simulink model "simulink_flightgear_control_trim_wind_5"  (R2023a)
settings: Solver=VariableStepAuto  StartTime=0  StopTime=inf  FixedStep=0.1  RelTol=1e-3
values from neighbouring files (symbols this model uses):
  alpha = -5:0.1:25    [Boeing747model.m]
  alpha1 = 0:0.1:14    [Boeing747model.m]
  alpha2 = -5:0.1:25    [Boeing747model.m]
  alpha3 = -5:0.1:17    [Boeing747model.m]
  beta = -15:0.1:15    [Boeing747model.m]
  CL = 0:0.01:1.4    [Boeing747model.m]
  da = 0:1:20    [Boeing747model.m]
  dr = [0 5 10 15 20 25]    [Boeing747model.m]
  EPR_ = 0:0.1:1.8    [Boeing747model.m]    (also in engine.m)
  flap = [0 10 20 25 30]    [Boeing747model.m]
  high1 = 0:10000:40000    [Boeing747model.m]
  high2 = 0:20000:40000    [Boeing747model.m]
  high3 = [0 15000 25000 35000 40000]    [Boeing747model.m]    (also in engine.m)
  high4 = [0 10000 20000 40000]    [Boeing747model.m]
  interp_result = table2array(resultTable(:,2:end))    [Boeing747model.m]
  interp_result_mach = 0:0.1:0.9    [Boeing747model.m]
  interp_result_N1 = 80:5:110    [Boeing747model.m]
  m2ft = 3.280839895013    (= 3.28083989501)    [Boeing747model.m]    (also in engine.m)
  mach = 0:0.02:0.9    [Boeing747model.m]    (also in engine.m)
  mach1 = [0 0.3 0.5 0.7 0.8 0.84 0.86 0.88 0.9]    [Boeing747model.m]
  mach2 = [0 0.3 0.5 0.7 0.8 0.9]    [Boeing747model.m]
  mach3 = [0 0.1 0.3 0.5 0.6 0.7 0.8 0.9]    [Boeing747model.m]    (also in engine.m = [0 0.1 0.3 0.5  0.7 0.8 0.9])
  mach5 = [0 0.6 0.8 0.85 0.9]    [Boeing747model.m]
  mach6 = [0 0.6 0.8 0.9]    [Boeing747model.m]
  mach7 = [0 0.3 0.5 0.74 0.8 0.84 0.86 0.88 0.9]    [Boeing747model.m]
  mach8 = [0 0.3 0.5 0.74 0.8 0.84 0.86 0.88 0.9]    [Boeing747model.m]
  model = 'simulink_flightgear_control_trim_wind_5'    [traimcode.m]
  ms2kts = 1.943844492609    (= 1.94384449261)    [Boeing747model.m]    (also in engine.m)
  powerangle_ = 0:1:130    [Boeing747model.m]    (also in engine.m)
  T = [-45 0 60 120]    [Boeing747model.m]    (also in engine.m)
  V_E = 0:20:250    [Boeing747model.m]
undefined symbols (not defined in the file or in its folder): Earth, F, ft, Light, m, MIL, Model, Newton, P3DAERO, Raphson, Receive, s, Send, Unit, WGS84, Wind
libraries: simulink_extras x115, aerolibconvert2 x16, simulink x4, aerolibfltsims x3, shared6dof x1, aerolibasang x1, aerolibtransform2 x1, aerolibatmos2 x1, aerolibobsolete x1, aerolibwind2 x1
(part 2 of 5)

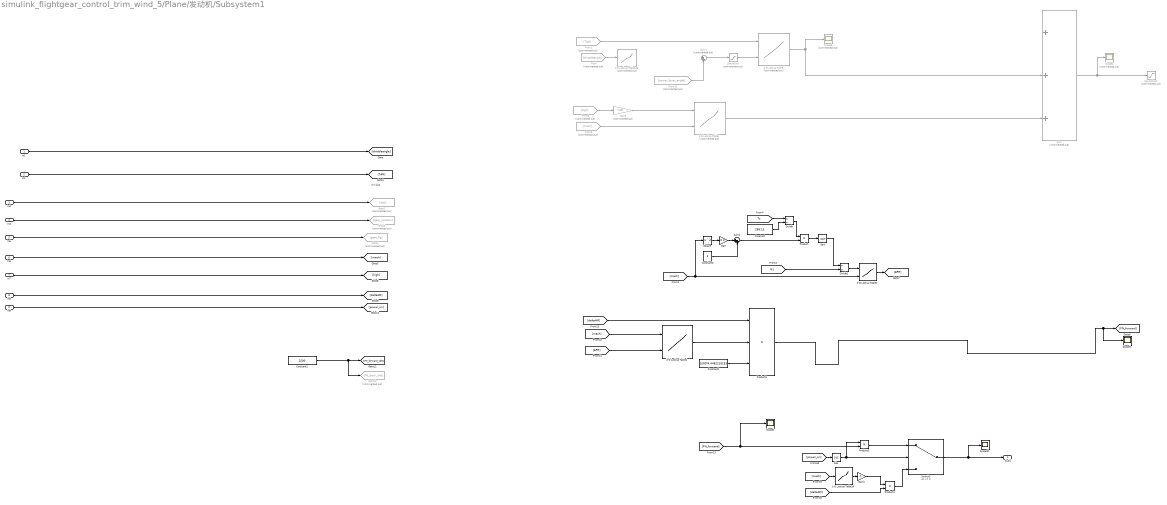
== system simulink_flightgear_control_trim_wind_5/Plane/发动机/Subsystem1 ==
  note: 华氏温度
  In1 : Inport
  In2 : Inport  Port=2
  In3 : Inport  Port=3
  In4 : Inport  Port=4
  In5 : Inport  Port=5
  In6 : Inport  Port=6
  In7 : Inport  Port=7
  In8 : Inport  Port=8
  In9 : Inport  Port=9
  1-D Lookup Table106 : Lookup_n-D  Commented=on  NumberOfTableDimensions=1  BreakpointsForDimension1=P3DAERO.powerangle(1,:)  Table=P3DAERO.powerangle(2,:)  InternalRulePriority=Speed  RndMeth=Simplest
  1-D Lookup Table14 : Lookup_n-D  NumberOfTableDimensions=1  BreakpointsForDimension1=P3DAERO.FD_engine(1,:)  Table=P3DAERO.FD_engine(2,:)  InternalRulePriority=Speed  RndMeth=Simplest
  2-D Lookup Table : Lookup_n-D  Commented=on  BreakpointsForDimension1=T  BreakpointsForDimension2=powerangle_  Table=P3DAERO.tam  InternalRulePriority=Speed  RndMeth=Simplest
      settings: InputPortMap=u0,u1
  2-D Lookup Table1 : Lookup_n-D  Commented=on  BreakpointsForDimension1=high3  BreakpointsForDimension2=mach  Table=P3DAERO.EPR_decay  InternalRulePriority=Speed  RndMeth=Simplest
      settings: InputPortMap=u0,u1
  2-D Lookup Table2 : Lookup_n-D  BreakpointsForDimension1=interp_result_N1  BreakpointsForDimension2=interp_result_mach  Table=interp_result  InternalRulePriority=Speed  RndMeth=Simplest
      settings: InputPortMap=u0,u1
  2-D Lookup Table4 : Lookup_n-D  BreakpointsForDimension1=mach3  BreakpointsForDimension2=EPR_  Table=P3DAERO.FN_deltaAM  InternalRulePriority=Speed  RndMeth=Simplest
      settings: InputPortMap=u0,u1
  Abs : Abs  SaturateOnIntegerOverflow=off
  Constant : Constant  Value=288.15
  Constant1 : Constant  Value=1000*4.4482216153
  Constant2 : Constant  Value=2500
  Constant3 : Constant
  Divide : Product  Inputs=*/
  Divide1 : Product  Inputs=/*
  From : From  Commented=on  GotoTag=throttleangle
  From1 : From  Commented=on  GotoTag=TAM
  From10 : From  Commented=on  GotoTag=power_lever_angle
  From5 : From  Commented=on  GotoTag=mach
  From6 : From  Commented=on  GotoTag=high
  Gain : Gain  Gain=0.2
  Gain1 : Gain  Gain=-1
  Gain3 : Gain  Commented=on  Gain=m2ft
  Goto13 : Goto  Commented=on  GotoTag=FN_back_idle
  Goto2 : Goto  Commented=on  GotoTag=site
  Goto3 : Goto  Commented=on  GotoTag=gear_position
  Goto4 : Goto  Commented=on  GotoTag=gear_hg
  Product : Product
  Product4 : Product
  Product5 : Product
  Product6 : Product  Inputs=3
  Saturation : Saturate  Commented=on  UpperLimit=130  LowerLimit=0
  Saturation2 : Saturate  Commented=on  UpperLimit=1.7  LowerLimit=1
  Scope1 : Scope
  Scope11 : Scope
  Scope2 : Scope  Commented=on
  Scope3 : Scope
  Scope8 : Scope  Commented=on
  Sqrt : Sqrt
  Square : Math  Operator=square
  Sum : Sum  Commented=on  Inputs=+++
  Sum1 : Sum  Commented=on  Inputs=|++
  Sum2 : Sum  Inputs=|++
  Switch3 : Switch  Criteria=u2 ~= 0  SaturateOnIntegerOverflow=off  InputSameDT=off
  Out1 : Outport
  wires:
  From/1 -> 1-D Lookup Table106/1
  In2/1 -> [TAM]
  In1/1 -> [throttleangle]
  In5/1 -> Goto4/1
  In3/1 -> Goto2/1
  In4/1 -> Goto3/1
  In6/1 -> [mach]
  In8/1 -> [deltaAM]
  In7/1 -> [high]
  In9/1 -> [power_on]
  From1/1 -> 2-D Lookup Table/1
  From6/1 -> Gain3/1
  Gain3/1 -> 2-D Lookup Table1/1
  From5/1 -> 2-D Lookup Table1/2
  [deltaAM] -> Product6/1
  [EPR] -> 2-D Lookup Table4/2
  2-D Lookup Table4/1 -> Product6/2
  [mach] -> 2-D Lookup Table4/1
  Constant1/1 -> Product6/3
  Saturation/1 -> 2-D Lookup Table/2
  Constant2/1 -> [FN_forward_idle], Goto13/1
  Sum1/1 -> Saturation/1
  Product6/1 -> Scope3/1, [FN_forward]
  2-D Lookup Table/1 -> Sum/2, Scope8/1
  Sum/1 -> Saturation2/1, Scope2/1
  [FN_forward] -> Scope1/1, Product5/2
  Product5/1 -> Switch3/1
  Product4/1 -> Switch3/3
  [power_on] -> Abs/1
  [deltaAM] -> Product4/2
  Switch3/1 -> Scope11/1, Out1/1
  Abs/1 -> Product5/1, Switch3/2
  1-D Lookup Table14/1 -> Gain1/1
  Gain1/1 -> Product4/1
  [mach] -> 1-D Lookup Table14/1
  From10/1 -> Sum1/2
  2-D Lookup Table1/1 -> Sum/3
  Sqrt/1 -> Divide1/1
  Divide/1 -> Product/1
  [N1] -> Divide1/2
  Divide1/1 -> 2-D Lookup Table2/1
  Square/1 -> Gain/1
  Constant3/1 -> Sum2/2
  [Ts] -> Divide/1
  Sum2/1 -> Product/2
  Constant/1 -> Divide/2
  Gain/1 -> Sum2/1
  2-D Lookup Table2/1 -> [EPR]
  Product/1 -> Sqrt/1
  [mach] -> Square/1, 2-D Lookup Table2/2

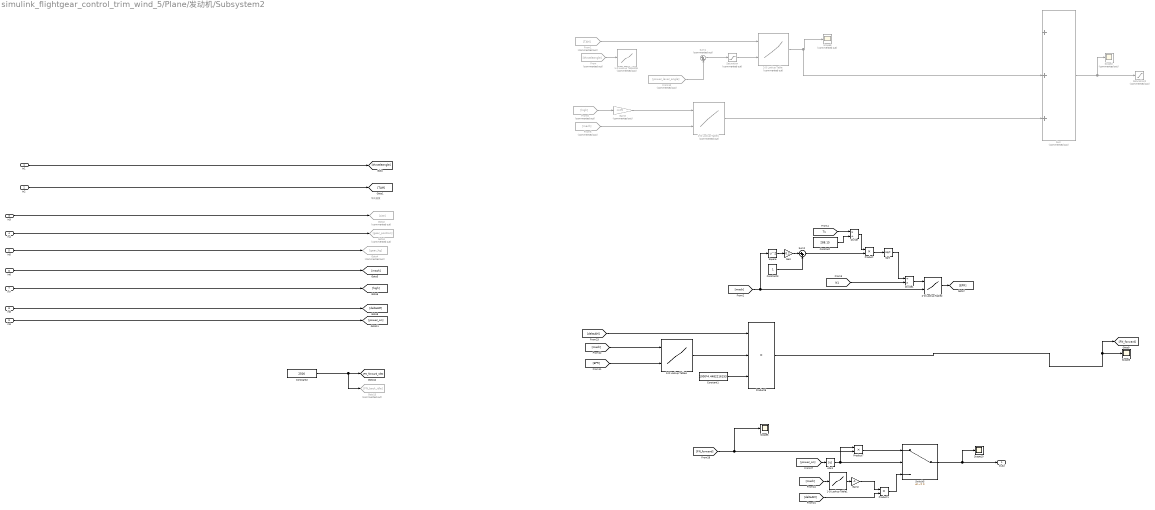
== system simulink_flightgear_control_trim_wind_5/Plane/发动机/Subsystem2 ==
  note: 华氏温度
  In1 : Inport
  In2 : Inport  Port=2
  In3 : Inport  Port=3
  In4 : Inport  Port=4
  In5 : Inport  Port=5
  In6 : Inport  Port=6
  In7 : Inport  Port=7
  In8 : Inport  Port=8
  In9 : Inport  Port=9
  1-D Lookup Table1 : Lookup_n-D  NumberOfTableDimensions=1  BreakpointsForDimension1=P3DAERO.FD_engine(1,:)  Table=P3DAERO.FD_engine(2,:)  InternalRulePriority=Speed  RndMeth=Simplest
  1-D Lookup Table106 : Lookup_n-D  Commented=on  NumberOfTableDimensions=1  BreakpointsForDimension1=P3DAERO.powerangle(1,:)  Table=P3DAERO.powerangle(2,:)  InternalRulePriority=Speed  RndMeth=Simplest
  2-D Lookup Table : Lookup_n-D  Commented=on  BreakpointsForDimension1=T  BreakpointsForDimension2=powerangle_  Table=P3DAERO.tam  InternalRulePriority=Speed  RndMeth=Simplest
      settings: InputPortMap=u0,u1
  2-D Lookup Table1 : Lookup_n-D  Commented=on  BreakpointsForDimension1=high3  BreakpointsForDimension2=mach  Table=P3DAERO.EPR_decay  InternalRulePriority=Speed  RndMeth=Simplest
      settings: InputPortMap=u0,u1
  2-D Lookup Table2 : Lookup_n-D  BreakpointsForDimension1=interp_result_N1  BreakpointsForDimension2=interp_result_mach  Table=interp_result  InternalRulePriority=Speed  RndMeth=Simplest
      settings: InputPortMap=u0,u1
  2-D Lookup Table4 : Lookup_n-D  BreakpointsForDimension1=mach3  BreakpointsForDimension2=EPR_  Table=P3DAERO.FN_deltaAM  InternalRulePriority=Speed  RndMeth=Simplest
      settings: InputPortMap=u0,u1
  Abs1 : Abs  SaturateOnIntegerOverflow=off
  Constant : Constant  Value=288.15
  Constant1 : Constant  Value=1000*4.4482216153
  Constant2 : Constant  Value=2500
  Constant3 : Constant
  Divide : Product  Inputs=*/
  Divide1 : Product  Inputs=/*
  From : From  Commented=on  GotoTag=throttleangle
  From1 : From  Commented=on  GotoTag=TAM
  From10 : From  Commented=on  GotoTag=power_lever_angle
  From5 : From  Commented=on  GotoTag=mach
  From6 : From  Commented=on  GotoTag=high
  Gain : Gain  Gain=0.2
  Gain2 : Gain  Gain=-1
  Gain3 : Gain  Commented=on  Gain=m2ft
  Goto13 : Goto  Commented=on  GotoTag=FN_back_idle
  Goto2 : Goto  Commented=on  GotoTag=site
  Goto3 : Goto  Commented=on  GotoTag=gear_position
  Goto4 : Goto  Commented=on  GotoTag=gear_hg
  Product : Product
  Product1 : Product
  Product6 : Product  Inputs=3
  Product7 : Product
  Saturation : Saturate  Commented=on  UpperLimit=130  LowerLimit=0
  Saturation2 : Saturate  Commented=on  UpperLimit=1.7  LowerLimit=1
  Scope10 : Scope
  Scope2 : Scope  Commented=on
  Scope3 : Scope
  Scope5 : Scope
  Scope8 : Scope  Commented=on
  Sqrt : Sqrt
  Square : Math  Operator=square
  Sum : Sum  Commented=on  Inputs=+++
  Sum1 : Sum  Commented=on  Inputs=|++
  Sum2 : Sum  Inputs=|++
  Switch5 : Switch  Criteria=u2 ~= 0  SaturateOnIntegerOverflow=off  InputSameDT=off
  Out2 : Outport
  wires:
  From/1 -> 1-D Lookup Table106/1
  In2/1 -> [TAM]
  In1/1 -> [throttleangle]
  In5/1 -> Goto4/1
  In3/1 -> Goto2/1
  In4/1 -> Goto3/1
  In6/1 -> [mach]
  In8/1 -> [deltaAM]
  In7/1 -> [high]
  In9/1 -> [power_on]
  From1/1 -> 2-D Lookup Table/1
  From6/1 -> Gain3/1
  Gain3/1 -> 2-D Lookup Table1/1
  From5/1 -> 2-D Lookup Table1/2
  [deltaAM] -> Product6/1
  [EPR] -> 2-D Lookup Table4/2
  2-D Lookup Table4/1 -> Product6/2
  [mach] -> 2-D Lookup Table4/1
  Constant1/1 -> Product6/3
  Saturation/1 -> 2-D Lookup Table/2
  Constant2/1 -> [FN_forward_idle], Goto13/1
  Sum1/1 -> Saturation/1
  Product6/1 -> [FN_forward], Scope3/1
  2-D Lookup Table/1 -> Sum/2, Scope8/1
  Sum/1 -> Saturation2/1, Scope2/1
  [FN_forward] -> Scope5/1, Product7/2
  Product7/1 -> Switch5/1
  Product1/1 -> Switch5/3
  [power_on] -> Abs1/1
  [deltaAM] -> Product1/2
  Switch5/1 -> Scope10/1, Out2/1
  Abs1/1 -> Product7/1, Switch5/2
  1-D Lookup Table1/1 -> Gain2/1
  Gain2/1 -> Product1/1
  [mach] -> 1-D Lookup Table1/1
  From10/1 -> Sum1/2
  2-D Lookup Table1/1 -> Sum/3
  Sqrt/1 -> Divide1/1
  Divide/1 -> Product/1
  [N1] -> Divide1/2
  Divide1/1 -> 2-D Lookup Table2/1
  Square/1 -> Gain/1
  Constant3/1 -> Sum2/2
  [Ts] -> Divide/1
  Sum2/1 -> Product/2
  Constant/1 -> Divide/2
  Gain/1 -> Sum2/1
  2-D Lookup Table2/1 -> [EPR]
  Product/1 -> Sqrt/1
  [mach] -> Square/1, 2-D Lookup Table2/2

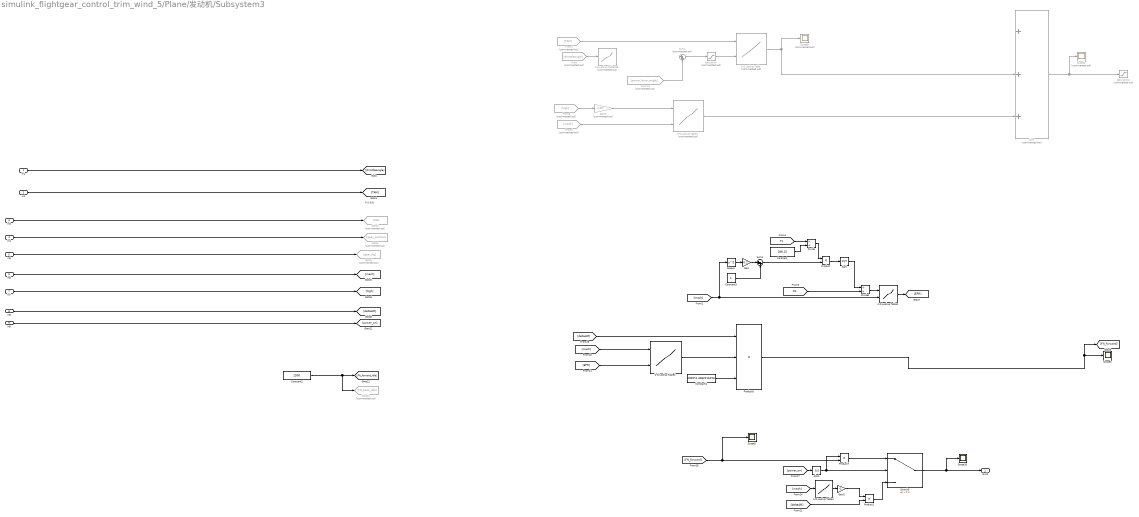
== system simulink_flightgear_control_trim_wind_5/Plane/发动机/Subsystem3 ==
  note: 华氏温度
  In1 : Inport
  In2 : Inport  Port=2
  In3 : Inport  Port=3
  In4 : Inport  Port=4
  In5 : Inport  Port=5
  In6 : Inport  Port=6
  In7 : Inport  Port=7
  In8 : Inport  Port=8
  In9 : Inport  Port=9
  1-D Lookup Table1 : Lookup_n-D  NumberOfTableDimensions=1  BreakpointsForDimension1=P3DAERO.FD_engine(1,:)  Table=P3DAERO.FD_engine(2,:)  InternalRulePriority=Speed  RndMeth=Simplest
  1-D Lookup Table106 : Lookup_n-D  Commented=on  NumberOfTableDimensions=1  BreakpointsForDimension1=P3DAERO.powerangle(1,:)  Table=P3DAERO.powerangle(2,:)  InternalRulePriority=Speed  RndMeth=Simplest
  2-D Lookup Table : Lookup_n-D  Commented=on  BreakpointsForDimension1=T  BreakpointsForDimension2=powerangle_  Table=P3DAERO.tam  InternalRulePriority=Speed  RndMeth=Simplest
      settings: InputPortMap=u0,u1
  2-D Lookup Table1 : Lookup_n-D  Commented=on  BreakpointsForDimension1=high3  BreakpointsForDimension2=mach  Table=P3DAERO.EPR_decay  InternalRulePriority=Speed  RndMeth=Simplest
      settings: InputPortMap=u0,u1
  2-D Lookup Table2 : Lookup_n-D  BreakpointsForDimension1=interp_result_N1  BreakpointsForDimension2=interp_result_mach  Table=interp_result  InternalRulePriority=Speed  RndMeth=Simplest
      settings: InputPortMap=u0,u1
  2-D Lookup Table4 : Lookup_n-D  BreakpointsForDimension1=mach3  BreakpointsForDimension2=EPR_  Table=P3DAERO.FN_deltaAM  InternalRulePriority=Speed  RndMeth=Simplest
      settings: InputPortMap=u0,u1
  Abs1 : Abs  SaturateOnIntegerOverflow=off
  Constant : Constant  Value=288.15
  Constant1 : Constant  Value=1000*4.4482216153
  Constant2 : Constant  Value=2500
  Constant3 : Constant
  Divide : Product  Inputs=*/
  Divide1 : Product  Inputs=/*
  From : From  Commented=on  GotoTag=throttleangle
  From1 : From  Commented=on  GotoTag=TAM
  From10 : From  Commented=on  GotoTag=power_lever_angle
  From5 : From  Commented=on  GotoTag=mach
  From6 : From  Commented=on  GotoTag=high
  Gain : Gain  Gain=0.2
  Gain2 : Gain  Gain=-1
  Gain3 : Gain  Commented=on  Gain=m2ft
  Goto13 : Goto  Commented=on  GotoTag=FN_back_idle
  Goto2 : Goto  Commented=on  GotoTag=site
  Goto3 : Goto  Commented=on  GotoTag=gear_position
  Goto4 : Goto  Commented=on  GotoTag=gear_hg
  Product : Product
  Product1 : Product
  Product6 : Product  Inputs=3
  Product7 : Product
  Saturation : Saturate  Commented=on  UpperLimit=130  LowerLimit=0
  Saturation1 : Saturate  Commented=on  UpperLimit=1.7  LowerLimit=1
  Scope10 : Scope
  Scope2 : Scope  Commented=on
  Scope3 : Scope
  Scope5 : Scope
  Scope8 : Scope  Commented=on
  Sqrt : Sqrt
  Square : Math  Operator=square
  Sum : Sum  Commented=on  Inputs=+++
  Sum1 : Sum  Commented=on  Inputs=|++
  Sum2 : Sum  Inputs=|++
  Switch5 : Switch  Criteria=u2 ~= 0  SaturateOnIntegerOverflow=off  InputSameDT=off
  Out2 : Outport
  wires:
  From/1 -> 1-D Lookup Table106/1
  In2/1 -> [TAM]
  In1/1 -> [throttleangle]
  In5/1 -> Goto4/1
  In3/1 -> Goto2/1
  In4/1 -> Goto3/1
  In6/1 -> [mach]
  In8/1 -> [deltaAM]
  In7/1 -> [high]
  In9/1 -> [power_on]
  From1/1 -> 2-D Lookup Table/1
  From6/1 -> Gain3/1
  Gain3/1 -> 2-D Lookup Table1/1
  From5/1 -> 2-D Lookup Table1/2
  [deltaAM] -> Product6/1
  [EPR] -> 2-D Lookup Table4/2
  2-D Lookup Table4/1 -> Product6/2
  [mach] -> 2-D Lookup Table4/1
  Constant1/1 -> Product6/3
  Saturation/1 -> 2-D Lookup Table/2
  Constant2/1 -> [FN_forward_idle], Goto13/1
  Sum1/1 -> Saturation/1
  Product6/1 -> [FN_forward], Scope3/1
  2-D Lookup Table/1 -> Sum/2, Scope8/1
  Sum/1 -> Saturation1/1, Scope2/1
  [FN_forward] -> Scope5/1, Product7/2
  Product7/1 -> Switch5/1
  Product1/1 -> Switch5/3
  [power_on] -> Abs1/1
  [deltaAM] -> Product1/2
  Switch5/1 -> Scope10/1, Out2/1
  Abs1/1 -> Product7/1, Switch5/2
  1-D Lookup Table1/1 -> Gain2/1
  Gain2/1 -> Product1/1
  [mach] -> 1-D Lookup Table1/1
  From10/1 -> Sum1/2
  2-D Lookup Table1/1 -> Sum/3
  Sqrt/1 -> Divide1/1
  Divide/1 -> Product/1
  [N1] -> Divide1/2
  Divide1/1 -> 2-D Lookup Table2/1
  Square/1 -> Gain/1
  Constant3/1 -> Sum2/2
  [Ts] -> Divide/1
  Sum2/1 -> Product/2
  Constant/1 -> Divide/2
  Gain/1 -> Sum2/1
  2-D Lookup Table2/1 -> [EPR]
  Product/1 -> Sqrt/1
  [mach] -> Square/1, 2-D Lookup Table2/2

== system simulink_flightgear_control_trim_wind_5/Plane/大气环境/风场_地面坐标系 ==
  Alt_Rel : Inport
  Vb* : Inport  Port=2
  Vgx : Inport  Port=3
  Add : Sum  Inputs=+++
  Atan2 : Trigonometry  Operator=atan2
  Compare To Constant : simulink/Logic and Bit Operations/Compare To Constant  relop=>=  const=Wind.Total.Act_Vb  OutDataTypeStr=uint8
  Constant : Constant  Value=[1 0 0;0 1 0;0 0 1]
  Constant3 : Constant  Value=Wind.Turblence.Strength
  Demux : Demux  Outputs=2
  Product1 : Product  Inputs=3
  Product{2..9} (8 alike) : Product
  Selector : Selector  InputPortWidth=3  IndexOptions=Index vector (dialog)  Indices=[2 1]  OutputSizes=1
  Subsystem : Subsystem
  Sum : Sum  Inputs=|++
  Wind_Constant_Act : Constant  Value=Wind.Constant.Act
  Wind_Custom_Act : Constant  Value=Wind.Custom.Act
  Wind_Gust_Act : Constant  Value=Wind.Gust.Act
  Wind_Turblence_Act : Constant  Value=Wind.Turblence.Act
  常值风 : Subsystem
  湍流 : aerolibwind2/Dryden Wind Turbulence Model  (Continuous (+q -r))  units=Metric (MKS)  spec=MIL-F-8785C  model=Continuous Dryden (+q +r)  W20=Wind.Constant.Vxy_Ground  Wdeg=Wind.Constant.Direction  TurbProb=10^-2 - Light  L_high=533.4  Wingspan=Model.b  ts=Wind.Turblence.SampleTime  Seed=[fix(rand(1,1)*25000), fix(rand(1,1)*25000+1), fix(rand(1,1)*25000+2), fix(rand(1,1)*25000+3)]  T_on=on
  自定义 : Subsystem
  阵风 : Subsystem
  V_Wind : Outport  VectorParamsAs1DForOutWhenUnconnected=off
  ω_Wind : Outport  Port=2  VectorParamsAs1DForOutWhenUnconnected=off
  Direction_Wind : Outport  Port=3  VectorParamsAs1DForOutWhenUnconnected=off
  wires:
  Wind_Custom_Act/1 -> Product8/2
  Product8/1 -> Add/3
  自定义/1(V_Wind_Custom) -> Product8/1
  Wind_Turblence_Act/1 -> Product2/1, Product1/2
  Wind_Gust_Act/1 -> Product7/2
  Wind_Constant_Act/1 -> Product4/2
  Demux/1 -> Atan2/1
  Demux/2 -> Atan2/2
  Selector/1 -> Demux/1
  Compare To Constant/1 -> Product9/1, Product6/1, Product5/1, Product3/1
  Atan2/1 -> Product3/2
  Subsystem/1(V_Wind) -> Sum/1
  Sum/1 -> Product5/2, Selector/1
  Product7/1 -> Add/2
  阵风/1(V_Wind_Gust) -> Product7/1
  Product4/1 -> Add/1
  Product1/1 -> Sum/2
  Product3/1 -> Direction_Wind/1
  Product2/1 -> Product6/2
  Constant3/1 -> Product1/1
  Product6/1 -> ω_Wind/1
  Product5/1 -> V_Wind/1
  Constant/1 -> 湍流/3
  常值风/1(V_Wind_Constant) -> Product4/1
  Vb*/1 -> Compare To Constant/1, 湍流/2
  湍流/2 -> Product2/2
  湍流/1 -> Product1/3
  Alt_Rel/1 -> 常值风/1(h(m)), 湍流/1
  Vgx/1 -> Subsystem/1(Vgx)
  Product9/1 -> Subsystem/2(WindSpeed)
  Add/1 -> Product9/2

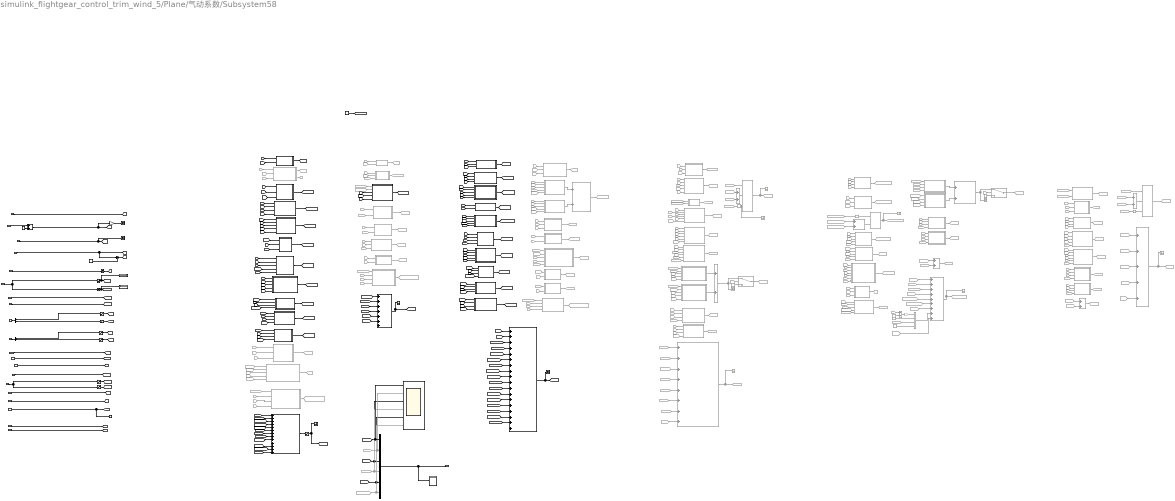
== system simulink_flightgear_control_trim_wind_5/Plane/气动系数/Subsystem58 ==
  note: degree
  note: 目前气动系数方向：
      | 升力向上为正
      | 阻力向后为正
      | 侧力向右为正
      | 俯仰力矩抬头为正
      | 滚转力矩右滚为正
      | 偏航力矩右偏为正
      | 升降舵下偏为正
      | 方向舵左偏为正
      | 副翼左侧向下右侧向右
      | 俯仰配平 前缘向上为正
  note: 输入单位:
      | 角度：弧度
      | 角速度：rad/s
      | 速度:mach
      | 舵面：rad
      | 襟翼：0-1
      | 高度：米
      | 重心：百分比
  note: 内侧升降舵偏转角度
  note: 平尾配平角度
  note: 迎角RAD+安装角
      | 安装角
  note: 外侧升降舵偏转角度
  note: 起落架时间控制系统
  note: Cl
  note: CL
  note: CN
  note: CC
  note: CD
  note: CM
  note: 襟翼角度
  note: CL
  In1 : Inport
  In2 : Inport  Port=2
  In3 : Inport  Port=3
  In4 : Inport  Port=4
  In5 : Inport  Port=5
  In6 : Inport  Port=6
  trim : Inport  Port=7
  In8 : Inport  Port=8
  aere_o : Inport  Port=9
  In10 : Inport  Port=10
  In11 : Inport  Port=11
  In12 : Inport  Port=12
  In13 : Inport  Port=13
  In14 : Inport  Port=14
  In15 : Inport  Port=15
  In16 : Inport  Port=16
  In17 : Inport  Port=17
  In18 : Inport  Port=18
  V_E : Inport  Port=19
  In20 : Inport  Port=20
  Bus Creator : BusCreator  Inputs=6
  Constant : Constant  Value=0.03490658504
  Constant1 : Constant  Commented=on  Value=25
  Constant10 : Constant  Commented=on  Value=27.3
  Constant15 : Constant  Commented=on  Value=0
  Constant2 : Constant  Commented=on  Value=0
  Constant3 : Constant  Commented=on  Value=195.7
  Constant4 : Constant  Value=4.58
  Constant5 : Constant  Value=0
  Demux : Demux  Outputs=2
  Demux1 : Demux  Outputs=2
  Display : Display
  Display1 : Display
  Display2 : Display
  Divide : Product  Commented=on  Inputs=***/
  From{6,10,14,47,53,68,72,84,125,140,144,171,176,182,188,192,201,212,215,217,232..233,237,239,241,248,252,255,266,282,284,286..287,289,301,309,313,323,326,334} (40 alike) : From  Commented=on  GotoTag=alpha
  From{16,44,101,142,187,228,265,383} (8 alike) : From  Commented=on  GotoTag=high_g
  From{7,11,43,48,58,75,77..78,85,124,130,137,143,145,173,175,190,193,195,200,203,208,210,213,218,221,231,240,254,260,263,270,291,300,304,307,325} (37 alike) : From  Commented=on  GotoTag=flap
  From128 : From  Commented=on  GotoTag=aerol_in_l
  From135 : From  Commented=on  GotoTag=aerol_in_r
  From{87,90,138..139,180,186,191,198,202,211,219,235,250..251,253,258,264,269,272,275,280,305..306} (23 alike) : From  Commented=on  GotoTag=mach
  From141 : From  Commented=on  GotoTag=Fm_ge
  From{65..66,73,146,177..178,189,196,222,267,285,335} (12 alike) : From  Commented=on  GotoTag=beta
  From{45,168,256,331} (4 alike) : From  Commented=on  GotoTag=left_aero
  From{46,169,257,332} (4 alike) : From  Commented=on  GotoTag=right_aero
  From170 : From  Commented=on  GotoTag=Fm_ge
  From172 : From  Commented=on  GotoTag=p
  From{74,179,234,288,310} (5 alike) : From  Commented=on  GotoTag=rudder_u
  From183 : From  Commented=on  GotoTag=Fm_ge
  From{69,184,238,290,314} (5 alike) : From  Commented=on  GotoTag=rudder_l
  From{95,185,324,336} (4 alike) : From  Commented=on  GotoTag=K
  From{194,197,199,206,209,236,259,261,268,271,276,283,311..312,328} (15 alike) : From  Commented=on  GotoTag=high
  From204 : From  Commented=on  GotoTag=V_E
  From205 : From  Commented=on  GotoTag=cg
  From207 : From  Commented=on  GotoTag=cg
  From214 : From  Commented=on  GotoTag=dot_CN_dot_beta_2
  From216 : From  Commented=on  GotoTag=r
  From220 : From  Commented=on  GotoTag=aerol_in_r
  From223 : From  Commented=on  GotoTag=dot_CN_dot_beta
  From224 : From  Commented=on  GotoTag=Fn_ge
  From225 : From  Commented=on  GotoTag=dot_CN_dot_beta_dian
  From226 : From  Commented=on  GotoTag=Fn_ge
  From227 : From  Commented=on  GotoTag=Fn_ge
  From229 : From  Commented=on  GotoTag=dot_beta
  From230 : From  Commented=on  GotoTag=p
  From242 : From  Commented=on  GotoTag=dot_CN_dot_p
  From243 : From  Commented=on  GotoTag=dot_CN_dot_r
  From244 : From  Commented=on  GotoTag=delta_CN_ai
  From245 : From  Commented=on  GotoTag=delta_CN_ao
  From246 : From  Commented=on  GotoTag=delata_CN_RU
  From247 : From  Commented=on  GotoTag=delata_CN_RL
  From249 : From  Commented=on  GotoTag=delata_CN_R
  From262 : From  Commented=on  GotoTag=p
  From273 : From  Commented=on  GotoTag=r
  From274 : From  Commented=on  GotoTag=dot_CC_dot_p
  From277 : From  Commented=on  GotoTag=dot_CC_dot_r
  From278 : From  Commented=on  GotoTag=dot_CC_dot_beta
  From279 : From  Commented=on  GotoTag=dot_Cl_dot_beta_1
  From281 : From  Commented=on  GotoTag=delata_CC_R
  From292 : From  Commented=on  GotoTag=delta_CC_25_RL
  From293 : From  Commented=on  GotoTag=delta_CC_25_RU
  From294 : From  Commented=on  GotoTag=dot_CC_dot_beta_1
  From295 : From  Commented=on  GotoTag=dot_CC_dot_beta_2
  From297 : From  Commented=on  GotoTag=F_c_beta_ge
  From298 : From  Commented=on  GotoTag=V_E
  From{76,299,302..303} (4 alike) : From  Commented=on  GotoTag=F_rho_ge
  From308 : From  Commented=on  GotoTag=dot_Cl_dot_beta_2
  From315 : From  Commented=on  GotoTag=dot_Cl_dot_beta
  From316 : From  Commented=on  GotoTag=doe_Cl_dot_p
  From317 : From  Commented=on  GotoTag=doe_Cl_dot_r
  From318 : From  Commented=on  GotoTag=delta_Cl_ai
  From319 : From  Commented=on  GotoTag=delta_Cl_ao
  From320 : From  Commented=on  GotoTag=delta_Cl_RL_25
  From321 : From  Commented=on  GotoTag=delta_Cl_RU_25
  From322 : From  Commented=on  GotoTag=r
  From329 : From  Commented=on  GotoTag=F_rho_beta_ge
  From330 : From  Commented=on  GotoTag=aerol_in_r
  From{337..343} (7 alike) : From  Commented=on  GotoTag=V  TagVisibility=global
  From353 : From  Commented=on  GotoTag=CN
  From355 : From  Commented=on  GotoTag=delata_CC_R
  From356 : From  Commented=on  GotoTag=cg
  From36 : From  Commented=on  GotoTag=CC
  From37 : From  Commented=on  GotoTag=Cl
  From379 : From  Commented=on  GotoTag=deltaCl_spoilers
  From381 : From  Commented=on  GotoTag=deltaCn_spoilers
  From382 : From  Commented=on  GotoTag=deltaCc_spoilers
  From41 : From  Commented=on  GotoTag=dot_CN_dot_beta_1
  From61 : From  Commented=on  GotoTag=Model_CG_Real_xyz  TagVisibility=global
  From81 : From  Commented=on  GotoTag=delta_FRL
  From82 : From  Commented=on  GotoTag=dot_CD_dot_delta
  From83 : From  Commented=on  GotoTag=CD_basic
  Gain1 : Gain  Gain=57.3
  Gain4 : Gain  Commented=on  Gain=0.01
  Goto100 : Goto  Commented=on  GotoTag=delta_Cl_ao
  Goto101 : Goto  Commented=on  GotoTag=dot_Cl_dot_beta_1
  Goto104 : Goto  Commented=on  GotoTag=k_ge_b
  Goto17 : Goto  Commented=on  GotoTag=F_rho_ge
  Goto18 : Goto  Commented=on  GotoTag=dot_CD_dot_delta
  Goto22 : Goto  Commented=on  GotoTag=deltaCL_Ao
  Goto25 : Goto  Commented=on  GotoTag=delta_CD_sideslip
  Goto28 : Goto  Commented=on  GotoTag=delta_CD_R_u
  Goto29 : Goto  Commented=on  GotoTag=delta_CL_landinggear
  Goto30 : Goto  Commented=on  GotoTag=delta_CL_ge
  Goto37 : Goto  Commented=on  GotoTag=delta_CD_R_l
  Goto38 : Goto  Commented=on  GotoTag=delta_CD_ge
  Goto39 : Goto  Commented=on  GotoTag=CD_basic
  Goto40 : Goto  Commented=on  GotoTag=delta_CD_landinggear
  Goto45 : Goto  Commented=on  GotoTag=delta_CM_25_R_u
  Goto50 : Goto  Commented=on  GotoTag=Fm_ge
  Goto51 : Goto  Commented=on  GotoTag=delta_CM_25_ao
  Goto52 : Goto  Commented=on  GotoTag=delta_CM_25_R_l
  Goto58 : Goto  Commented=on  GotoTag=delta_CM_25_landinggear
  Goto59 : Goto  Commented=on  GotoTag=delta_CM_25_ge
  Goto60 : Goto  Commented=on  GotoTag=delta_CM_25_sideslip
  Goto62 : Goto  Commented=on  GotoTag=delta_CM_25_ai
  Goto65 : Goto  Commented=on  GotoTag=Cl
  Goto66 : Goto  Commented=on  GotoTag=dot_Cl_dot_beta_2
  Goto67 : Goto  Commented=on  GotoTag=doe_Cl_dot_p
  Goto68 : Goto  Commented=on  GotoTag=dot_Cl_dot_beta
  Goto69 : Goto  Commented=on  GotoTag=doe_Cl_dot_r
  Goto70 : Goto  Commented=on  GotoTag=dot_CN_dot_beta_1
  Goto71 : Goto  Commented=on  GotoTag=dot_CN_dot_beta
  Goto72 : Goto  Commented=on  GotoTag=dot_CN_dot_p
  Goto73 : Goto  Commented=on  GotoTag=dot_CN_dot_r
  Goto74 : Goto  Commented=on  GotoTag=dot_CN_dot_beta_dian
  Goto75 : Goto  Commented=on  GotoTag=Fn_ge
  Goto78 : Goto  Commented=on  GotoTag=delta_CN_ai
  Goto79 : Goto  Commented=on  GotoTag=delata_CN_RU
  Goto80 : Goto  Commented=on  GotoTag=delata_CN_RL
  Goto81 : Goto  Commented=on  GotoTag=CN
  Goto82 : Goto  Commented=on  GotoTag=delata_CN_R
  Goto83 : Goto  Commented=on  GotoTag=delta_CN_ao
  Goto84 : Goto  Commented=on  GotoTag=dot_CN_dot_beta_2
  Goto85 : Goto  Commented=on  GotoTag=dot_CC_dot_p
  Goto86 : Goto  Commented=on  GotoTag=dot_CC_dot_beta_2
  Goto87 : Goto  Commented=on  GotoTag=CC
  Goto88 : Goto  Commented=on  GotoTag=dot_CC_dot_beta
  Goto89 : Goto  Commented=on  GotoTag=dot_CC_dot_r
  Goto90 : Goto  Commented=on  GotoTag=delta_CC_25_RU
  Goto91 : Goto  Commented=on  GotoTag=delta_CC_25_RL
  Goto92 : Goto  Commented=on  GotoTag=delata_CC_R
  Goto93 : Goto  Commented=on  GotoTag=F_c_beta_ge
  Goto94 : Goto  Commented=on  GotoTag=dot_CC_dot_beta_1
  Goto96 : Goto  Commented=on  GotoTag=delta_Cl_ai
  Goto97 : Goto  Commented=on  GotoTag=delta_Cl_RU_25
  Goto98 : Goto  Commented=on  GotoTag=delta_Cl_RL_25
  Goto99 : Goto  Commented=on  GotoTag=F_rho_beta_ge
  Product : Product  Commented=on
  Product1 : Product  Commented=on  Inputs=3
  Product3 : Product  Commented=on  Inputs=3
  Radians to Degrees1 : simulink_extras/Transformations/Radians to Degrees  Commented=on
      settings: LibrarySourceBlock=|
      | simulink/Plane/气动系数/Subsystem58/Radians
      | to Degrees1
  Radians to Degrees3 : simulink_extras/Transformations/Radians to Degrees  Commented=on
      settings: LibrarySourceBlock=|
      | simulink/Plane/气动系数/Subsystem58/Radians
      | to Degrees3
  Radians to Degrees4 : simulink_extras/Transformations/Radians to Degrees  Commented=on
      settings: LibrarySourceBlock=|
      | simulink/Plane/气动系数/Subsystem58/Radians
      | to Degrees4
  Saturation1 : Saturate  UpperLimit=0.26  LowerLimit=-0.436
  Saturation10 : Saturate  UpperLimit=0.26  LowerLimit=-0.436
  Saturation12 : Saturate  UpperLimit=33  LowerLimit=14
  Saturation14 : Saturate  UpperLimit=0.436  LowerLimit=-0.436
  Saturation16 : Saturate  UpperLimit=0.436  LowerLimit=-0.436
  Saturation3 : Saturate  UpperLimit=0.349  LowerLimit=-0.349
  Saturation4 : Saturate  UpperLimit=0.349  LowerLimit=-0.349
  Saturation6 : Saturate  UpperLimit=3  LowerLimit=-2
  Saturation8 : Saturate  UpperLimit=0.4  LowerLimit=-0.296
  Saturation9 : Saturate  UpperLimit=0.4  LowerLimit=-0.296
  Scope{,2..7,44} (8 alike) : Scope  Commented=on
  Scope{1,11..12,14,16,21} (6 alike) : Scope
  Scope10 : Scope  NumInputPorts=6
  Subsystem : Subsystem
  Subsystem1 : Subsystem
  Subsystem10 : Subsystem
  Subsystem12 : Subsystem  Commented=on
  Subsystem13 : Subsystem  Commented=on
  Subsystem14 : Subsystem
  Subsystem15 : Subsystem  Commented=on
  Subsystem16 : Subsystem  Commented=on
  Subsystem17 : Subsystem  Commented=on
  Subsystem18 : Subsystem  Commented=on
  Subsystem19 : Subsystem  Commented=on
  Subsystem2 : Subsystem
  Subsystem20 : Subsystem
  Subsystem21 : Subsystem
  Subsystem22 : Subsystem  Commented=on
  Subsystem23 : Subsystem  Commented=on
  Subsystem24 : Subsystem  Commented=on
  Subsystem25 : Subsystem  Commented=on
  Subsystem26 : Subsystem  Commented=on
  Subsystem27 : Subsystem  Commented=on
  Subsystem28 : Subsystem  Commented=on
  Subsystem29 : Subsystem  Commented=on
  Subsystem3 : Subsystem
  Subsystem30 : Subsystem
  Subsystem31 : Subsystem
  Subsystem32 : Subsystem
  Subsystem33 : Subsystem
  Subsystem34 : Subsystem
  Subsystem35 : Subsystem
  Subsystem36 : Subsystem
  Subsystem37 : Subsystem
  Subsystem38 : Subsystem  Commented=on
  Subsystem39 : Subsystem  Commented=on
  Subsystem4 : Subsystem
  Subsystem40 : Subsystem  Commented=on
  Subsystem41 : Subsystem  Commented=on
  Subsystem42 : Subsystem  Commented=on
  Subsystem43 : Subsystem  Commented=on
  Subsystem44 : Subsystem  Commented=on
  Subsystem45 : Subsystem  Commented=on
  Subsystem46 : Subsystem  Commented=on
  Subsystem47 : Subsystem  Commented=on
  Subsystem48 : Subsystem  Commented=on
  Subsystem49 : Subsystem  Commented=on
  Subsystem5 : Subsystem
  Subsystem50 : Subsystem  Commented=on
  Subsystem51 : Subsystem  Commented=on
  Subsystem52 : Subsystem  Commented=on
  Subsystem53 : Subsystem  Commented=on
  Subsystem54 : Subsystem  Commented=on
  Subsystem55 : Subsystem  Commented=on
  Subsystem56 : Subsystem  Commented=on
  Subsystem57 : Subsystem  Commented=on
  Subsystem58 : Subsystem  Commented=on
  Subsystem59 : Subsystem  Commented=on
  Subsystem6 : Subsystem
  Subsystem60 : Subsystem  Commented=on
  Subsystem61 : Subsystem  Commented=on
  Subsystem62 : Subsystem  Commented=on
  Subsystem63 : Subsystem  Commented=on
  Subsystem64 : Subsystem  Commented=on
  Subsystem65 : Subsystem  Commented=on
  Subsystem66 : Subsystem
  Subsystem67 : Subsystem  Commented=on
  Subsystem68 : Subsystem  Commented=on
  Subsystem69 : Subsystem  Commented=on
  Subsystem7 : Subsystem
  Subsystem8 : Subsystem  Commented=on
  Subsystem9 : Subsystem  Commented=on
  Sum{,1,3,6,8..9,18,25} (8 alike) : Sum  Commented=on
  Sum10 : Sum  Commented=on  Inputs=+++++++++
  Sum11 : Sum  Commented=on  Inputs=+++++
  Sum12 : Sum  Commented=on  Inputs=+-
  Sum13 : Sum  Inputs=|+-
  Sum2 : Sum  Inputs=+++++++++++++
  Sum22 : Sum  Inputs=++++++++++++++++++
  Sum4 : Sum  Inputs=+++++++
  Sum5 : Sum
  Sum7 : Sum  Commented=on  Inputs=++++++++
  Switch13 : Switch  Commented=on  Criteria=u2 ~= 0  Threshold=0.35  SaturateOnIntegerOverflow=off  InputSameDT=off
  Switch3 : Switch  Commented=on  Criteria=u2 ~= 0  Threshold=0.35  SaturateOnIntegerOverflow=off  InputSameDT=off
  Coefficients1 : Outport
  tag scope: V=global
  wires:
  In2/1 -> Sum5/1  "alpha"
  In17/1 -> [r]  "r"
  In6/1 -> Saturation8/1, Saturation9/1  "Elevators"
  In10/1 -> [dot_alpha]  "dot_alpha"
  Saturation12/1 -> [cg]
  In13/1 -> [beta]  "beta"
  Saturation8/1 -> Display1/1, [delta_ei]
  In5/1 -> Saturation12/1  "cg"
  In8/1 -> [gear_position]  "gear_position"
  In1/1 -> [flap]  "flap"
  In11/1 -> [q]  "q"
  In16/1 -> [p]  "p"
  In3/1 -> Scope12/1, [mach]  "mach"
  Saturation16/1 -> [rudder_l]
  Saturation14/1 -> [rudder_u]
  In4/1 -> [high], Sum13/1  "high"
  trim/1 -> [delta_FRL]
  In14/1 -> Saturation14/1, Saturation16/1  "rudder"
  Saturation9/1 -> Display2/1, [delta_eo]
  In18/1 -> Scope16/1, [dot_beta]  "dot_beta"
  In12/1 -> [nz]  "nz"
  Constant/1 -> Sum5/2
  Sum5/1 -> Gain1/1, [alpha]
  V_E/1 -> [V_E]
  In20/1 -> [V]  "V"
  From208/1 -> Subsystem44/2(In2)
  From43/1 -> Subsystem58/3(In3)
  From177/1 -> Subsystem28/2(Radians in1)
  Sum18/1 -> Scope44/1, Switch3/1
  From215/1 -> Subsystem43/3(Radians in)
  [delta_eo] -> Subsystem37/4(Radians in)
  From184/1 -> Subsystem29/1(Radians in)
  [dot_CM_dot_delta_eo] -> Sum22/10
  From137/1 -> Subsystem24/3(In3)
  Subsystem28/1(Out1) -> Goto45/1
  [delta_CD_R_l] -> Sum4/5
  From11/1 -> Subsystem12/1(In1)
  Subsystem5/1(Out1) -> [dot_CL_dot_alpha_dian]
  From171/1 -> Subsystem27/4(Radians in)
  From81/1 -> Subsystem13/3(Radians in1)
  From68/1 -> Subsystem17/3(Radians in)
  From169/1 -> Subsystem27/5(Radians in1)
  Subsystem17/1(Out1) -> Goto38/1
  From83/1 -> Subsystem14/1(In1)
  [delta_CD_landinggear] -> Sum4/2
  Subsystem67/1(Out1) -> Goto29/1
  [delta_CD_ge] -> Sum4/3
  [flap] -> Subsystem14/3(In3)
  [delta_CD_R_u] -> Sum4/6
  Saturation6/1 -> [CL], Scope21/1
  From135/1 -> Subsystem24/4(Radians in1)
  [delta_CM_25_ai] -> Sum22/11
  [high] -> Subsystem1/3(In3)
  From130/1 -> Subsystem23/3(In3)
  [delta_CM_25_landinggear] -> Sum22/13
  [delta_CM_25_R_l] -> Sum22/16
  [delta_dot_CM_25_dot_alpha] -> Sum22/3
  From139/1 -> Subsystem24/1(In1)
  [alpha] -> Subsystem20/2(Radians in)
  From144/1 -> Subsystem25/3(Radians in)
  Subsystem20/1(Out1) -> [Cm_25_basic]
  [mach] -> Subsystem21/4(In4)
  [high] -> Subsystem35/2(In2)
  Subsystem30/1(Out1) -> [delta_dot_CM_25_dot_alpha]
  Subsystem33/1(Out1) -> [dot_CM_25_dot_q]
  [mach] -> Subsystem30/5(In5)
  [q] -> Subsystem33/3(In3)
  From128/1 -> Subsystem23/4(Radians in1)
  From77/1 -> Subsystem13/1(In1)
  [high] -> Subsystem34/4(In4)
  [flap] -> Subsystem1/1(In1)
  [delta_eo] -> Subsystem2/4(Radians in)
  From16/1 -> Subsystem22/1(In1)
  From182/1 -> Subsystem24/2(Radians in)
  [mach] -> Subsystem37/3(In3)
  Subsystem37/1(Out1) -> [dot_CM_dot_delta_eo]
  [mach] -> Subsystem34/5(In5)
  From125/1 -> Subsystem22/3(Radians in)
  From236/1 -> Subsystem41/1(In1)
  Subsystem18/1(Out1) -> Goto25/1
  From237/1 -> Subsystem41/3(Radians in)
  From212/1 -> Subsystem39/3(Radians in)
  From311/1 -> Subsystem59/1(In1)
  From302/1 -> Subsystem56/1(In1)
  From250/1 -> Subsystem39/4(In4)
  [dot_CL_dot_nz] -> Sum2/6
  Subsystem59/1(Out1) -> Goto97/1
  From87/1 -> Subsystem67/4(In4)
  From205/1 -> Subsystem40/3(In3)
  [CD_basic_real] -> Sum4/1
  [dot_CM_25_dot_nz] -> Sum22/7
  From82/1 -> Subsystem14/2(In2)
  From217/1 -> Subsystem45/3(Radians in)
  From95/1 -> Subsystem19/1(In1)
  From265/1 -> Subsystem8/1(In1)
  Subsystem45/1(Out1) -> Goto75/1
  [dot_CM_25_dot_q] -> Sum22/6
  [CL] -> Subsystem31/1(In1)
  Subsystem12/1(Out1) -> Goto39/1
  From251/1 -> Subsystem43/4(In4)
  From260/1 -> Subsystem43/2(In2)
  Sum4/1 -> [CD], Scope1/1
  From227/1 -> Subsystem48/1(In1)
  [high] -> Subsystem21/3(In3)
  Subsystem68/1(Out1) -> Goto96/1
  From240/1 -> Subsystem45/2(In2)
  [V_E] -> Subsystem7/3(In3)
  From290/1 -> Subsystem54/4(Radians in1)
  [mach] -> Subsystem66/3(In3)
  From272/1 -> Subsystem54/2(In2)
  From191/1 -> Subsystem65/4(In4)
  From314/1 -> Subsystem60/4(In4)
  Subsystem46/1(Out1) -> Goto78/1
  From268/1 -> Subsystem52/3(In3)
  From228/1 -> Subsystem49/1(In1)
  From249/1 -> Sum10/7
  From297/1 -> Product1/1
  From75/1 -> Subsystem18/1(In1)
  From242/1 -> Sum10/4
  From269/1 -> Subsystem53/2(In2)
  Subsystem3/1(Out1) -> [k_alpha]
  Subsystem41/1(Out1) -> Goto80/1
  From197/1 -> Subsystem65/3(In3)
  Sum/1 -> Product1/2
  From264/1 -> Subsystem52/4(In4)
  From222/1 -> Radians to Degrees1/1
  From266/1 -> Subsystem52/2(Radians in)
  [dot_CM_dot_delta_ei] -> Sum22/9
  Subsystem19/1(Out1) -> Goto40/1
  Subsystem34/1(Out1) -> [dot_CM_25_dot_nz]
  From286/1 -> Subsystem49/3(Radians in)
  From66/1 -> Subsystem16/1(Radians in)
  From318/1 -> Sum7/4
  From263/1 -> Subsystem50/1(In1)
  Subsystem9/1(Out1) -> Goto17/1
  From300/1 -> Switch3/2
  Subsystem49/1(Out1) -> Goto93/1
  From284/1 -> Subsystem51/4(Radians in)
  From124/1 -> Subsystem22/2(In2)
  From203/1 -> Subsystem56/3(In3)
  From326/1 -> Subsystem68/3(Radians in)
  From280/1 -> Subsystem51/2(In2)
  From270/1 -> Subsystem51/3(In3)
  From282/1 -> Subsystem50/2(Radians in)
  [CM] -> Scope10/5, Bus Creator/5
  From321/1 -> Sum7/7
  From14/1 -> Subsystem12/2(Radians in)
  From310/1 -> Subsystem59/4(In4)
  Subsystem51/1(Out1) -> Goto85/1
  [delta_CL_landinggear] -> Sum2/12
  Sum3/1 -> Switch13/1, Scope5/1
  From254/1 -> Switch13/2
  From141/1 -> Subsystem23/5(In5)
  Subsystem7/1(Out1) -> [dot_CL_dot_nz]
  From247/1 -> Sum8/2
  [flap] -> Subsystem20/1(In1)
  From69/1 -> Subsystem16/2(In2)
  From283/1 -> Subsystem50/3(In3)
  From206/1 -> Subsystem39/1(In1)
  Subsystem42/1(Out1) -> Goto74/1
  Radians to Degrees1/1 -> Product/1
  From329/1 -> Product3/1
  From195/1 -> Subsystem62/2(In2)
  Subsystem40/1(Out1) -> Goto84/1
  From331/1 -> Subsystem56/2(Radians in)
  From41/1 -> Sum1/1
  From231/1 -> Subsystem48/3(In3)
  From214/1 -> Sum1/2
  From243/1 -> Sum10/3
  Sum10/1 -> Scope/1, Goto81/1
  From220/1 -> Subsystem46/5(Radians in1)
  From78/1 -> Subsystem17/2(In2)
  [mach] -> Subsystem32/3(In3)
  From230/1 -> Subsystem43/1(In1)
  From170/1 -> Subsystem27/1(In1)
  From304/1 -> Subsystem52/1(In1)
  From335/1 -> Subsystem63/4(Radians in1)
  From194/1 -> Subsystem63/5(In5)
  From210/1 -> Subsystem40/1(In1)
  [high] -> Subsystem2/2(In2)
  Product1/1 -> Goto88/1
  [mach] -> Subsystem2/3(In3)
  From76/1 -> Subsystem58/1(In1)
  [delta_CM_25_R_u] -> Sum22/17
  From145/1 -> Subsystem26/1(In1)
  [high] -> Subsystem10/2(In2)
  From168/1 -> Subsystem27/2(In2)
  [delta_Cm_25] -> Sum22/2
  From334/1 -> Subsystem63/3(Radians in)
  Subsystem50/1(Out1) -> Goto94/1
  [flap] -> Subsystem21/1(In1)
  From224/1 -> Subsystem46/4(In4)
  From262/1 -> Subsystem51/1(In1)
  From337/1 -> Subsystem64/6(In6)
  [high] -> Subsystem30/4(In4)
  From235/1 -> Subsystem41/2(In2)
  From186/1 -> Subsystem63/1(In1)
  Radians to Degrees4/1 -> Product1/3
  Subsystem48/1(Out1) -> Sum3/2
  Subsystem35/1(Out1) -> [dot_CM_dot_delta]
  From325/1 -> Subsystem63/2(In2)
  Sum6/1 -> Product3/2
  Sum11/1 -> Scope2/1, Goto87/1
  [k_alpha] -> Subsystem66/1(In1)
  Subsystem16/1(Out1) -> Goto37/1
  From279/1 -> Sum6/1
  [delta_CM_25_ge] -> Sum22/14
  [flap] -> Subsystem34/2(In2)
  Subsystem/1(Out1) -> [CL_basic]
  Subsystem47/1(Out1) -> Sum3/1
  [k_alpha] -> Subsystem36/1(In1)
  Subsystem44/1(Out1) -> Goto73/1
  From211/1 -> Subsystem42/3(In3)
  From209/1 -> Subsystem42/2(In2)
  [alpha] -> Subsystem3/2(Radians in)
  Subsystem27/1(Out1) -> Goto51/1
  Subsystem14/1(Out1) -> [CD_basic_real]
  Subsystem65/1(Out1) -> Goto69/1
  From226/1 -> Subsystem47/1(In1)
  From299/1 -> Subsystem68/6(In6)
  [delta_CM_25_sideslip] -> Sum22/15
  [alpha] -> Subsystem4/1(Radians in)
  From285/1 -> Subsystem55/2(Radians in)
  From246/1 -> Sum8/1
  Subsystem15/1(Out1) -> Goto28/1
  From343/1 -> Subsystem52/6(In6)
  From219/1 -> Subsystem46/1(In1)
  [CL] -> Subsystem14/5(In5)
  Sum8/1 -> Goto82/1
  From276/1 -> Subsystem54/1(In1)
  From85/1 -> Subsystem19/2(In2)
  From255/1 -> Subsystem48/4(Radians in1)
  [delta_CM_25_ao] -> Sum22/12
  From173/1 -> Subsystem27/3(In3)
  [V_E] -> Subsystem21/2(In2)
  From176/1 -> Subsystem38/3(Radians in)
  From256/1 -> Subsystem47/2(Radians in)
  From339/1 -> Subsystem42/5(In5)
  [high] -> Subsystem37/2(In2)
  From287/1 -> Subsystem53/3(Radians in)
  From288/1 -> Subsystem53/4(Radians in1)
  From324/1 -> Subsystem55/1(In1)
  From223/1 -> Sum10/6
  From289/1 -> Subsystem54/3(Radians in)
  Subsystem38/1(Out1) -> Goto58/1
  Subsystem57/1(Out1) -> Sum18/2
  From259/1 -> Subsystem61/1(In1)
  [high] -> Subsystem66/2(In2)
  From200/1 -> Subsystem68/2(In2)
  From143/1 -> Subsystem25/2(In2)
  From341/1 -> Subsystem44/7(In7)
  From244/1 -> Sum10/2
  From313/1 -> Subsystem60/3(Radians in)
  [V] -> Subsystem33/4(In4)
  From234/1 -> Subsystem61/4(Radians in1)
  From53/1 -> Subsystem67/3(Radians in)
  Subsystem29/1(Out1) -> Goto52/1
  [dot_CL_dot_q] -> Sum2/5
  From239/1 -> Subsystem44/3(Radians in)
  Subsystem53/1(Out1) -> Goto90/1
  From291/1 -> Subsystem49/2(In2)
  From48/1 -> Subsystem8/2(In2)
  From273/1 -> Subsystem52/5(In5)
  From278/1 -> Sum11/1
  From187/1 -> Subsystem45/1(In1)
  [V] -> Subsystem32/5(In5)
  From336/1 -> Subsystem69/1(In1)
  From74/1 -> Subsystem15/2(In2)
  [V] -> Subsystem6/5(In5)
  From340/1 -> Subsystem43/5(In5)
  From261/1 -> Subsystem44/4(In4)
  Subsystem55/1(Out1) -> Goto86/1
  [mach] -> Subsystem35/3(In3)
  Sum9/1 -> Goto92/1
  [mach] -> Subsystem33/2(In2)
  From275/1 -> Subsystem50/4(In4)
  Subsystem43/1(Out1) -> Goto72/1
  [high] -> Subsystem33/1(In1)
  [high] -> Subsystem7/4(In4)
  [dot_alpha] -> Subsystem5/1(In1)
  [dot_CL_dot_alpha_dian] -> Sum2/4
  From140/1 -> Subsystem23/2(Radians in)
  Subsystem58/1(Out1) -> Goto22/1
  [high] -> Subsystem32/2(In2)
  [nz] -> Subsystem7/1(In1)
  [CL_basic] -> Sum2/1
  From58/1 -> Subsystem67/2(In2)
  From202/1 -> Subsystem68/1(In1)
  [flap] -> Subsystem3/1(In1)
  From322/1 -> Subsystem65/5(In5)
  Sum25/1 -> Goto62/1
  [flap] -> Subsystem4/2(In2)
  From101/1 -> Subsystem62/1(In1)
  From61/1 -> Subsystem67/1(In1)
  Subsystem62/1(Out1) -> Goto99/1
  [flap] -> Subsystem30/2(In2)
  From330/1 -> Subsystem68/5(In5)
  From178/1 -> Subsystem29/2(Radians in1)
  From277/1 -> Sum11/3
  From204/1 -> Subsystem56/5(In5)
  From216/1 -> Subsystem44/6(In6)
  [cg] -> Subsystem32/1(u)
  Subsystem54/1(Out1) -> Goto91/1
  From248/1 -> Subsystem40/2(Radians in)
  Subsystem21/1(Out1) -> [delta_Cm_25]
  From312/1 -> Subsystem60/1(In1)
  From229/1 -> Subsystem42/4(In4)
  Sum1/1 -> Product/2
  Subsystem13/1(Out1) -> Goto18/1
  [delta_ei] -> Subsystem36/4(Radians in)
  Product/1 -> Scope7/1, Goto71/1
  [mach] -> Subsystem1/4(In4)
  From308/1 -> Sum6/2
  [CL] -> Scope10/3, Bus Creator/3
  [mach] -> Subsystem6/3(In3)
  From281/1 -> Sum11/4
  From37/1 -> Scope10/4, Bus Creator/4
  From292/1 -> Sum9/1
  From353/1 -> Scope10/6, Bus Creator/6
  From305/1 -> Subsystem59/2(In2)
  From36/1 -> Scope10/2, Bus Creator/2
  Subsystem39/1(Out1) -> Goto70/1
  Constant15/1 -> Switch13/3
  From213/1 -> Subsystem39/2(In2)
  From383/1 -> Subsystem9/1(In1)
  [cg] -> Subsystem6/1(u)
  From218/1 -> Subsystem46/2(In2)
  Subsystem8/1(Out1) -> Goto30/1
  [mach] -> Subsystem5/2(In2)
  [q] -> Subsystem6/4(In4)
  From303/1 -> Subsystem57/1(In1)
  From46/1 -> Subsystem58/5(Radians in2)
  From252/1 -> Subsystem47/4(Radians in1)
  From271/1 -> Subsystem53/1(In1)
  [k_alpha] -> Subsystem2/1(In1)
  [Cm_25_basic] -> Sum22/1
  From7/1 -> Subsystem9/2(In2)
  Bus Creator/1 -> Display/1, Coefficients1/1  "parameter"
  Subsystem26/1(Out1) -> Goto60/1
  Subsystem10/1(Out1) -> [dot_CL_dot_delta_ei]
  Subsystem4/1(Out1) -> [delta_dot_CL_dot_alpha]
  From245/1 -> Sum10/1
  [alpha] -> Subsystem/2(Radians in)
  Subsystem1/1(Out1) -> [delta_CL]
  Subsystem25/1(Out1) -> Goto59/1
  From241/1 -> Subsystem46/3(Radians in)
  [delta_FRL] -> Subsystem35/4(Radians in)
  From185/1 -> Subsystem38/1(In1)
  [deltaCL_Ao] -> Sum2/11
  [mach] -> Subsystem10/3(In3)
  [delta_CL_ge] -> Sum2/13
  From45/1 -> Subsystem58/2(Radians in)
  From257/1 -> Subsystem48/2(Radians in)
  [mach] -> Subsystem36/3(In3)
  [mach] -> Subsystem14/4(In4)
  Subsystem23/1(Out1) -> Sum25/1
  [V_E] -> Subsystem4/3(In3)
  Subsystem52/1(Out1) -> Goto89/1
  From253/1 -> Subsystem44/5(In5)
  From190/1 -> Subsystem65/1(In1)
  From274/1 -> Sum11/2
  [delta_CD_sideslip] -> Sum4/4
  Subsystem61/1(Out1) -> Goto79/1
  From225/1 -> Sum10/5
  From233/1 -> Subsystem61/3(Radians in)
  From188/1 -> Subsystem65/2(Radians in)
  From175/1 -> Subsystem38/2(In2)
  From320/1 -> Sum7/6
  [dot_alpha] -> Subsystem32/4(In4)
  From309/1 -> Subsystem59/3(Radians in)
  Subsystem36/1(Out1) -> [dot_CM_dot_delta_ei]
  [high] -> Subsystem6/2(In2)
  From189/1 -> Radians to Degrees3/1
  From294/1 -> Sum/1
  From138/1 -> Subsystem23/1(In1)
  Sum7/1 -> Scope3/1, Goto65/1
  Subsystem6/1(Out1) -> [dot_CL_dot_q]
  [mach] -> Subsystem7/5(In5)
  [alpha] -> Subsystem30/1(Radians in)
  From295/1 -> Sum/2
  From198/1 -> Subsystem64/4(In4)
  Sum2/1 -> Saturation6/1
  From90/1 -> Subsystem19/4(In4)
  [cg] -> Subsystem31/2(In2)
  From201/1 -> Subsystem56/4(Radians in1)
  [flap] -> Subsystem7/2(In2)
  Subsystem32/1(Out1) -> [dot_CM_25_dot_alpha_dian]
  [V] -> Subsystem5/3(In3)
  [delta_FRL] -> Subsystem66/4(Radians in)
  [k_alpha] -> Subsystem10/1(In1)
  From84/1 -> Subsystem19/3(Radians in)
  From179/1 -> Subsystem28/1(Radians in)
  From267/1 -> Radians to Degrees4/1
  From258/1 -> Subsystem61/2(In2)
  From192/1 -> Subsystem64/2(Radians in)
  From298/1 -> Subsystem57/5(In5)
  [k_alpha] -> Subsystem35/1(In1)
  From319/1 -> Sum7/5
  From332/1 -> Subsystem57/2(Radians in)
  From183/1 -> Subsystem24/5(In5)
  From338/1 -> Subsystem65/6(In6)
  [V_E] -> Subsystem1/2(In2)
  From44/1 -> Subsystem17/1(In1)
  [dot_CM_25_dot_alpha_dian] -> Sum22/5
  [mach] -> Subsystem4/5(In5)
  [V_E] -> Subsystem30/3(In3)
  Subsystem24/1(Out1) -> Sum25/2
  Radians to Degrees3/1 -> Scope4/1, Product3/3
  Switch13/1 -> Goto83/1
  [high] -> Subsystem4/4(In4)
  From65/1 -> Subsystem15/1(Radians in)
  Subsystem56/1(Out1) -> Sum18/1
  [dot_CM_dot_delta] -> Sum22/8
  From6/1 -> Subsystem9/3(Radians in)
  Constant2/1 -> Switch3/3
  From196/1 -> Subsystem69/2(Radians in)
  From317/1 -> Sum7/3
  From307/1 -> Subsystem57/3(In3)
  From193/1 -> Subsystem64/1(In1)
  From142/1 -> Subsystem25/1(In1)
  [delta_ei] -> Subsystem10/4(Radians in)
  From146/1 -> Subsystem26/2(Radians in)
  [V_E] -> Subsystem34/3(In3)
  From323/1 -> Subsystem62/3(Radians in)
  From306/1 -> Subsystem60/2(In2)
  From199/1 -> Subsystem64/3(In3)
  [mach] -> Subsystem/3(In3)
  [CM_CL_CG_25] -> Sum22/4
  From10/1 -> Subsystem58/4(Radians in1)
  From315/1 -> Sum7/1
  [CD] -> Scope10/1, Bus Creator/1
  Product3/1 -> Scope6/1, Goto68/1
  [nz] -> Subsystem34/1(In1)
  From72/1 -> Subsystem13/2(Radians in)
  [delta_dot_CL_dot_alpha] -> Sum2/3
  [high] -> Subsystem36/2(In2)
  From73/1 -> Subsystem18/2(Radians in)
  From221/1 -> Subsystem47/3(In3)
  Subsystem31/1(Out1) -> [CM_CL_CG_25]
  [k_alpha] -> Subsystem37/1(In1)
  From342/1 -> Subsystem51/5(In5)
  Subsystem60/1(Out1) -> Goto98/1
  [flap] -> Subsystem/1(In1)
  From293/1 -> Sum9/2
  Subsystem22/1(Out1) -> Goto50/1
  From47/1 -> Subsystem8/3(Radians in)
  From301/1 -> Subsystem57/4(Radians in1)
  Subsystem2/1(Out1) -> [dot_CL_dot_delta_eo]
  Subsystem66/1(Out1) -> [dot_CL_dot_delta]
  [dot_CL_dot_delta_eo] -> Sum2/9
  [dot_CL_dot_delta_ei] -> Sum2/8
  [delta_CL] -> Sum2/2
  From316/1 -> Sum7/2
  Subsystem69/1(Out1) -> Goto66/1
  Sum22/1 -> Scope14/1, [CM]
  From238/1 -> Subsystem41/4(Radians in1)
  From180/1 -> Subsystem38/4(In4)
  From207/1 -> Subsystem44/1(u)
  From172/1 -> Subsystem64/5(In5)
  [dot_CL_dot_delta] -> Sum2/7
  Switch3/1 -> Goto100/1
  From232/1 -> Subsystem42/1(Radians in)
  From328/1 -> Subsystem68/4(In4)
  [mach] -> Subsystem20/3(In3)
  Gain1/1 -> Scope11/1
  Subsystem64/1(Out1) -> Goto67/1
  Subsystem63/1(Out1) -> Goto101/1
  From356/1 -> Sum12/1
  Constant1/1 -> Sum12/2
  Sum12/1 -> Gain4/1
  Gain4/1 -> Divide/1
  From355/1 -> Divide/3
  Constant3/1 -> Divide/4
  Constant10/1 -> Divide/2
  Divide/1 -> Sum10/8
  Demux/1 -> Saturation10/1
  Demux/2 -> Saturation1/1
  In15/1 -> Demux1/1  "ai"
  Saturation3/1 -> [aerol_in_l]
  Demux1/2 -> Saturation4/1
  Saturation4/1 -> [aerol_in_r]
  Saturation10/1 -> [left_aero]
  Demux1/1 -> Saturation3/1
  aere_o/1 -> Demux/1
  Saturation1/1 -> [right_aero]
  Subsystem9/2(Out2) -> Goto104/1
  From379/1 -> Sum7/8
  From381/1 -> Sum10/9
  From382/1 -> Sum11/5
  Sum13/1 -> [high_g]
  Constant4/1 -> Sum13/2
  Constant5/1 -> [K]

== system simulink_flightgear_control_trim_wind_5/Plane/参数计算/Subsystem1/Subsystem ==
  Vb : Inport
  Demux1 : Demux  Outputs=3
      settings: DisplayOption=none
  Terminator : Terminator
  w : Outport  VectorParamsAs1DForOutWhenUnconnected=off
  u : Outport  Port=2  VectorParamsAs1DForOutWhenUnconnected=off
  wires:
  Demux1/2 -> Terminator/1
  Vb/1 -> Demux1/1
  Demux1/1 -> u/1
  Demux1/3 -> w/1

== system simulink_flightgear_control_trim_wind_5/Plane/参数计算/Subsystem1/Subsystem1 ==
  Vb : Inport
  Demux1 : Demux  Outputs=3
      settings: DisplayOption=none
  Terminator : Terminator
  Terminator1 : Terminator
  v : Outport  VectorParamsAs1DForOutWhenUnconnected=off
  wires:
  Demux1/3 -> Terminator1/1
  Demux1/1 -> Terminator/1
  Demux1/2 -> v/1
  Vb/1 -> Demux1/1

== system simulink_flightgear_control_trim_wind_5/Plane/参数计算/Subsystem1/Subsystem2 ==
  Vb : Inport
  Demux1 : Demux  Outputs=3
  Product1 : Product  RndMeth=Zero
  Product2 : Product  RndMeth=Zero
  Product3 : Product  RndMeth=Zero
  Sum : Sum  Inputs=+++
  u²+v²+w² : Outport  VectorParamsAs1DForOutWhenUnconnected=off
  wires:
  Demux1/1 -> Product1/1, Product1/2
  Product1/1 -> Sum/1
  Sum/1 -> u²+v²+w²/1
  Demux1/3 -> Product3/1, Product3/2
  Vb/1 -> Demux1/1
  Product2/1 -> Sum/2
  Demux1/2 -> Product2/2, Product2/1
  Product3/1 -> Sum/3

== system simulink_flightgear_control_trim_wind_5/Plane/参数计算/航迹角/Subsystem ==
  Vg : Inport
  Demux1 : Demux  Outputs=3
      settings: DisplayOption=none
  Terminator : Terminator
  Vy : Outport  VectorParamsAs1DForOutWhenUnconnected=off
  Vx : Outport  Port=2  VectorParamsAs1DForOutWhenUnconnected=off
  wires:
  Vg/1 -> Demux1/1
  Demux1/1 -> Vx/1
  Demux1/3 -> Terminator/1
  Demux1/2 -> Vy/1

== system simulink_flightgear_control_trim_wind_5/Plane/参数计算/航迹角/Subsystem1 ==
  Vg : Inport
  Demux1 : Demux  Outputs=3
      settings: DisplayOption=none
  Terminator : Terminator
  Terminator1 : Terminator
  Vz : Outport  VectorParamsAs1DForOutWhenUnconnected=off
  wires:
  Demux1/1 -> Terminator/1
  Vg/1 -> Demux1/1
  Demux1/3 -> Vz/1
  Demux1/2 -> Terminator1/1
